simulink model "DFN_LPF_diff"  (R2023a)
settings: Solver=VariableStepAuto  StartTime=0.0  StopTime=5  RelTol=1e-3
undefined symbols (not defined in the file or in its folder): DiscIntNeverNeededParam
libraries: simulink x1
settings Model: Creator=tshintai  LastModifiedBy=tshintai
settings SolverCC: AlgebraicLoopSolver=TrustRegion
settings OptimizationCC: ReuseModelBlockBuffer=off
settings DebuggingCC: UnconnectedInputMsg=warning  UnconnectedOutputMsg=warning  UnconnectedLineMsg=warning
settings ModelReferenceCC: EnableRefExpFcnMdlSchedulingChecks=on
settings RTWCC: DLArmComputeVersion=19.05

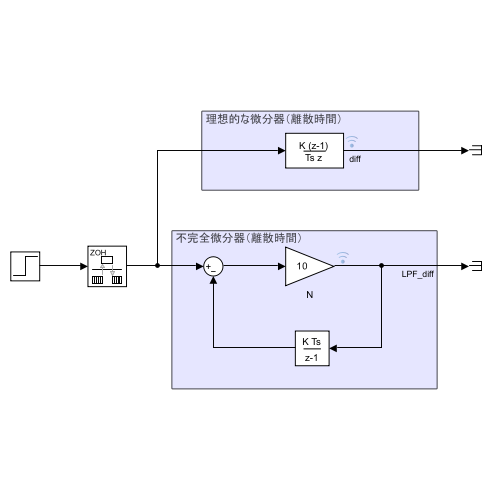
[thumbnail: Simulink's stored preview of the top-level diagram]
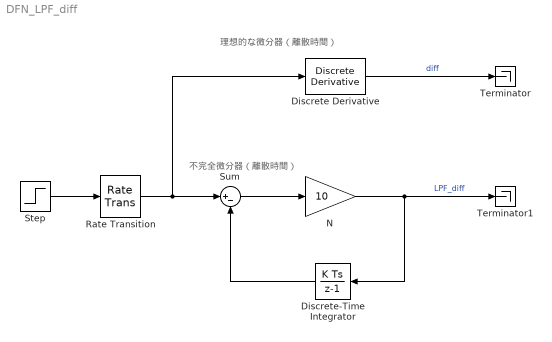
== system DFN_LPF_diff ==
  note: 不完全微分器（離散時間）
  note: 理想的な微分器（離散時間）
  Discrete Derivative : simulink/Discrete/Discrete Derivative  gainval=1.0  ICPrevScaledInput=0.0  OutMin=[]  OutMax=[]  OutDataType=fixdt(1, 16)  OutScaling=2^-10  DoSatur=off
  Discrete-Time Integrator : DiscreteIntegrator  SampleTime=-1  ICPrevOutput=DiscIntNeverNeededParam  ICPrevScaledInput=DiscIntNeverNeededParam
  N : Gain  Gain=10
  Rate Transition : RateTransition  OutPortSampleTime=0.01
  Step : Step  SampleTime=0
  Sum : Sum  Inputs=|+-
  Terminator : Terminator
  Terminator1 : Terminator
  wires:
  Step/1 -> Rate Transition/1
  Sum/1 -> N/1
  Discrete-Time Integrator/1 -> Sum/2
  Rate Transition/1 -> Discrete Derivative/1, Sum/1
  N/1 -> Terminator1/1, Discrete-Time Integrator/1  "LPF_diff"
  Discrete Derivative/1 -> Terminator/1  "diff"
